simulink model "SHRKIM002_Dubins"  (R2026a)
settings: Solver=VariableStepAuto  StopTime=inf  MaxStep=0.04
InitFcn:
  | % Robot params
  | r_w = (67.60 / 2) / 1000; % wheel radius in m
  | d = (83 + 12.5 + 12.5) / 1000; % wheel centre-centre distance (width)
  | a = 33.275 / 1000; % IMU to wheel axle distance
  | 
  | % Motor params
  | k = 0.0192;
  | tau = 0.1718;
  | k_bodge = 3;
  | tau_bodge = 0.4;
  | 
  | noiseScalar = 1;
  | 
  | %control loop update rate
  | dt_loop = 0.02;
  | dt_sim = 0.005;
  | dt_plot = 0.1;
  | 
  | waypoint_matrix = centerlineTrack('SaoPaulo.csv');
model workspace (MAT data in the model file):
  d = Simulink.Parameter
  d.Value = 0.108
  d.Complexity = 'real'
  d.Dimensions = [1 1]
  d.DataType = 'auto'
  dphi_limit = Simulink.Parameter
  dphi_limit.Value = 9.72
  dphi_limit.Complexity = 'real'
  dphi_limit.Dimensions = [1 1]
  dphi_limit.DataType = 'double'
  dt_sim = Simulink.Parameter
  dt_sim.Value = 0.02
  dt_sim.Complexity = 'real'
  dt_sim.Dimensions = [1 1]
  dt_sim.DataType = 'auto'
  l_robot = Simulink.Parameter
  l_robot.Value = 0.103
  l_robot.Complexity = 'real'
  l_robot.Dimensions = [1 1]
  l_robot.DataType = 'auto'
  m_robot = Simulink.Parameter
  m_robot.Value = 0.5
  m_robot.Complexity = 'real'
  m_robot.Dimensions = [1 1]
  m_robot.DataType = 'auto'
  mpc_comp = mpc
  mpc_comp.Ts = 0.02
  mpc_comp.PredictionHorizon = 25
  mpc_comp.ControlHorizon = 2
  mpc_comp.Model.Plant = ss
  mpc_comp.Model.Plant.InputName_ = ["Robot Navigation & Control/Mux(1)"; "Robot Navigation & Control/Mux(2)"]
  mpc_comp.Model.Plant.InputGroup_.Manipulated = [1 2]
  mpc_comp.Model.Plant.OutputName_ = ["Plant Error Dynamics/1"; "Plant Error Dynamics/2"]
  mpc_comp.Model.Plant.OutputGroup_.Measured = [1 2]
  mpc_comp.Model.Plant.Name_ = 'Linearization at model initial condition'
  mpc_comp.Model.Plant.IOSize_ = [2 2]
  mpc_comp.Model.Plant.Data_ = ltipack.ssdata
  mpc_comp.Model.Plant.Data_.StateName = ["Integrator"; "Integrator1"]
  mpc_comp.Model.Plant.Data_.StatePath = ["SHRKIM002_FYP/Robot Navigation & Control/Plant Error Dynamics/Integrator"; "SHRKIM002_FYP/Robot Navigation & Control/Plant Error Dynamics/Integrator1"]
  mpc_comp.Model.Plant.Data_.a = [1  0; 0.004  1]
  mpc_comp.Model.Plant.Data_.c = [0  1; 1  0]
  mpc_comp.Model.Plant.Data_.dx0 = [0; 0]
  mpc_comp.Model.Plant.Data_.x0 = [0; 0]
  mpc_comp.Model.Plant.Data_.b = [-0.00625925925926  0.00625925925926; -1.25185185185e-05  1.25185185185e-05]
  mpc_comp.Model.Plant.Data_.d = [0  0; 0  0]
  mpc_comp.Model.Plant.Data_.u0 = [0; 0]
  mpc_comp.Model.Plant.Data_.y0 = [0; 0]
  mpc_comp.Model.Plant.Data_.Delay.Input = [0; 0]
  mpc_comp.Model.Plant.Data_.Delay.Output = [0; 0]
  mpc_comp.Model.Plant.Data_.Delay.Internal = []
  mpc_comp.Model.Plant.Data_.Ts = 0.02
  mpc_comp.Model.Disturbance = []
  mpc_comp.Model.Noise = []
  mpc_comp.Model.Nominal.X = [0; 0]
  mpc_comp.Model.Nominal.DX = [0; 0]
  mpc_comp.Model.Nominal.U = [0; 0]
  mpc_comp.Model.Nominal.Y = [0; 0]
  mpc_comp.ManipulatedVariables(1).Min = -9.72
  mpc_comp.ManipulatedVariables(1).Max = 9.72
  mpc_comp.ManipulatedVariables(1).MinECR = 0
  mpc_comp.ManipulatedVariables(1).MaxECR = 0
  mpc_comp.ManipulatedVariables(1).RateMin = -Inf
  mpc_comp.ManipulatedVariables(1).RateMax = Inf
  mpc_comp.ManipulatedVariables(1).RateMinECR = 0
  mpc_comp.ManipulatedVariables(1).RateMaxECR = 0
  mpc_comp.ManipulatedVariables(1).Target = 'nominal'
  mpc_comp.ManipulatedVariables(1).Name = 'Robot Navigation & Control/Mux(1)'
  mpc_comp.ManipulatedVariables(1).Units = ''
  mpc_comp.ManipulatedVariables(1).ScaleFactor = 1
  mpc_comp.ManipulatedVariables(1).Type = 'continuous'
  mpc_comp.ManipulatedVariables(2).Min = -9.72
  mpc_comp.ManipulatedVariables(2).Max = 9.72
  mpc_comp.ManipulatedVariables(2).MinECR = 0
  mpc_comp.ManipulatedVariables(2).MaxECR = 0
  mpc_comp.ManipulatedVariables(2).RateMin = -Inf
  mpc_comp.ManipulatedVariables(2).RateMax = Inf
  mpc_comp.ManipulatedVariables(2).RateMinECR = 0
  mpc_comp.ManipulatedVariables(2).RateMaxECR = 0
  mpc_comp.ManipulatedVariables(2).Target = 'nominal'
  mpc_comp.ManipulatedVariables(2).Name = 'Robot Navigation & Control/Mux(2)'
  mpc_comp.ManipulatedVariables(2).Units = ''
  mpc_comp.ManipulatedVariables(2).ScaleFactor = 1
  mpc_comp.ManipulatedVariables(2).Type = 'continuous'
  mpc_comp.OutputVariables(1).Min = -0.235
  mpc_comp.OutputVariables(1).Max = 0.235
  mpc_comp.OutputVariables(1).MinECR = 1
  mpc_comp.OutputVariables(1).MaxECR = 1
  mpc_comp.OutputVariables(1).Name = 'Plant Error Dynamics/1'
  mpc_comp.OutputVariables(1).Units = ''
  mpc_comp.OutputVariables(1).ScaleFactor = 1
  mpc_comp.OutputVariables(2).Min = -0.5236
  mpc_comp.OutputVariables(2).Max = 0.5236
  mpc_comp.OutputVariables(2).MinECR = 1
  mpc_comp.OutputVariables(2).MaxECR = 1
  mpc_comp.OutputVariables(2).Name = 'Plant Error Dynamics/2'
  mpc_comp.OutputVariables(2).Units = ''
  mpc_comp.OutputVariables(2).ScaleFactor = 1
  mpc_comp.Weights.ManipulatedVariables = [0.05 0.05]
  mpc_comp.Weights.ManipulatedVariablesRate = [0.1 0.1]
  mpc_comp.Weights.OutputVariables = [0.7 0.5]
  mpc_comp.Weights.ECR = 100000
  mpc_comp.Optimizer.OptimizationType = 'QP'
  mpc_comp.Optimizer.Solver = 'active-set'
  mpc_comp.Optimizer.SolverOptions = mpc.solver.options.qp.ActiveSet
  mpc_comp.Optimizer.SolverOptions.SolverName = 'ActiveSet'
  mpc_comp.Optimizer.MinOutputECR = 0
  mpc_comp.Optimizer.UseSuboptimalSolution = 0
  mpc_comp.Optimizer.CustomSolver = 0
  mpc_comp.Optimizer.CustomSolverCodeGen = 0
  mpc_comp.History = [2026 10 10 3 50 16.273]
  mpc_comp.MPCData = mpcdata
  mpc_comp.MPCData.IsDirty = 1
  mpc_comp.MPCData.Ts = 0.02
  mpc_comp.MPCData.p = 25
  mpc_comp.MPCData.m = 2
  mpc_comp.MPCData.UseActiveSetSolver = 1
  mpc_comp.MPCData.UseSuboptimalSolution = 0
  mpc_comp.MPCData.CustomSolver = 0
  mpc_comp.MPCData.CustomSolverCodeGen = 0
  mpc_comp.MPCData.IsCustomEstimation = 1
  mpc_comp.MPCData.Uscale = [1; 1]
  mpc_comp.MPCData.Yscale = [1; 1]
  mpc_comp.MPCData.mvindex = [1; 2]
  mpc_comp.MPCData.myindex = [1; 2]
  mpc_comp.MPCData.ASOptions.MaxIterations = 120
  mpc_comp.MPCData.ASOptions.ConstraintTolerance = 1e-06
  mpc_comp.MPCData.ASOptions.UseWarmStart = 1
  mpc_comp.MPCData.IPOptions.MaxIterations = 50
  mpc_comp.MPCData.IPOptions.ConstraintTolerance = 1e-06
  mpc_comp.MPCData.IPOptions.OptimalityTolerance = 1e-06
  mpc_comp.MPCData.IPOptions.ComplementarityTolerance = 1e-08
  mpc_comp.MPCData.IPOptions.StepTolerance = 1e-08
  mpc_comp.MPCData.ADOptions.AbsoluteTolerance = 0.001
  mpc_comp.MPCData.ADOptions.RelativeTolerance = 0.001
  mpc_comp.MPCData.ADOptions.MaxIterations = 1000
  mpc_comp.MPCData.ADOptions.RelaxationParameter = 1.6
  mpc_comp.MPCData.ADOptions.PenaltyParameter = 0.1
  mpc_comp.MPCData.ADOptions.StepSize = 1e-06
  mpc_comp.MPCData.ADOptions.PrimalInfeasibilityTolerance = 0.0001
  mpc_comp.MPCData.ADOptions.DualInfeasibilityTolerance = 0.0001
  mpc_comp.MPCData.ADOptions.EnablePolish = 0
  mpc_comp.MPCData.ADOptions.PolishRegularization = 1e-06
  mpc_comp.MPCData.ADOptions.PolishTolerance = 1e-08
  mpc_comp.MPCData.ADOptions.PolishMaxIterations = 3
  mpc_comp.MPCData.MIQPOptions.MaxIterations = 1000
  mpc_comp.MPCData.MIQPOptions.ConstraintTolerance = 1e-06
  mpc_comp.MPCData.MIQPOptions.UseWarmStart = 0
  mpc_comp.MPCData.MIQPOptions.DiscreteConstraintTolerance = 1e-06
  mpc_comp.MPCData.MIQPOptions.RoundingAtRootNode = 1
  mpc_comp.MPCData.MIQPOptions.MaxPendingNodes = 1000
  mpc_comp.IsEmpty = 0
  mpc_comp.OldOVIntegrator = {[]; []}
  mpc_comp.EstGain = 'custom'
  mpc_comp.OutDistModel = tf
  mpc_comp.OutDistModel.IOSize_ = [2 1]
  mpc_comp.OutDistModel.Data_ = ltipack.tfdata
  mpc_comp.OutDistModel.Data_.num = {0; 0}
  mpc_comp.OutDistModel.Data_.den = {1; 1}
  mpc_comp.OutDistModel.Data_.Delay.Input = 0
  mpc_comp.OutDistModel.Data_.Delay.Output = [0; 0]
  mpc_comp.OutDistModel.Data_.Delay.IO = [0; 0]
  mpc_comp.OutDistModel.Data_.Ts = 0
  mpc_comp.Version = '26.1'
  nlobj : nlmpc (value not decoded)
  no_points = Simulink.Parameter
  no_points.Value = 3000
  no_points.Complexity = 'real'
  no_points.Dimensions = [1 1]
  no_points.DataType = 'auto'
  r_w = Simulink.Parameter
  r_w.Value = 0.0338
  r_w.Complexity = 'real'
  r_w.Dimensions = [1 1]
  r_w.DataType = 'double'
  rho_min = Simulink.Parameter
  rho_min.Value = 0.2
  rho_min.Complexity = 'real'
  rho_min.Dimensions = [1 1]
  rho_min.DataType = 'auto'
  robot_half_w = Simulink.Parameter
  robot_half_w.Value = 0.065
  robot_half_w.Complexity = 'real'
  robot_half_w.Dimensions = [1 1]
  robot_half_w.DataType = 'auto'
  sample_f = Simulink.Parameter
  sample_f.Value = 50
  sample_f.Complexity = 'real'
  sample_f.Dimensions = [1 1]
  sample_f.DataType = 'auto'
  track_width = Simulink.Parameter
  track_width.Value = 0.6
  track_width.Complexity = 'real'
  track_width.Dimensions = [1 1]
  track_width.DataType = 'auto'
  waypoint_gain = Simulink.Parameter
  waypoint_gain.Value = 0.025
  waypoint_gain.Complexity = 'real'
  waypoint_gain.Dimensions = [1 1]
  waypoint_gain.DataType = 'auto'
values from neighbouring files (symbols this model uses):
  dphi_limit = 9.72    [controlNMPC.m]
undefined symbols (not defined in the file or in its folder): DiscIntNeverNeededParam
libraries: simulink x12, dspstat3 x6, slpidlib x2, mpclib x2, robotalgslib x1
(part 1 of 2)
settings Model: Creator=dylan  LastModifiedBy=Kim
settings SolverCC: DecoupledContinuousIntegration=on
settings SimscapeCC: SimscapeNominalValues="[{\"value\":\"1\",\"unit\":\"A\"},{\"value\":\"1\",\"unit\":\"bar\"},{\"value\":\"1\",\"unit\":\"cm^2\"},{\"value\":\"1\",\"unit\":\"cm^3/s\"},{\"value\":\"1\",\"unit\":\"kJ/kg\"},{\"value\":\"1\",\"unit\":\"kW\"},{\"value\":\"1\",\"unit\":\"l\"},{\"value\":\"1\",\"unit\":\"N\"},{\"value\":\"1\",\"unit\":\"N*m\"},{\"value\":\"1\",\"unit\":\"V\"}]"  SimscapeLogType=none  SimscapeLogDataHistory=5000.0

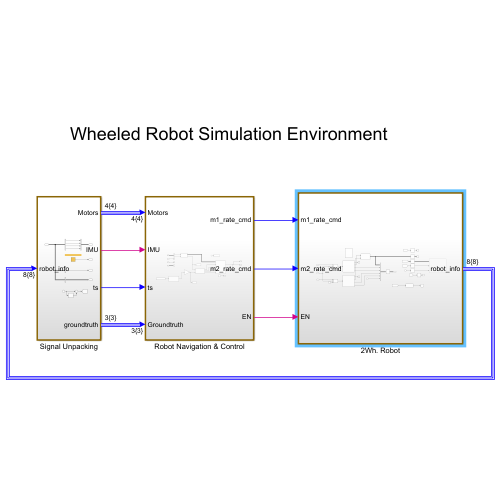
[thumbnail: Simulink's stored preview of the top-level diagram]
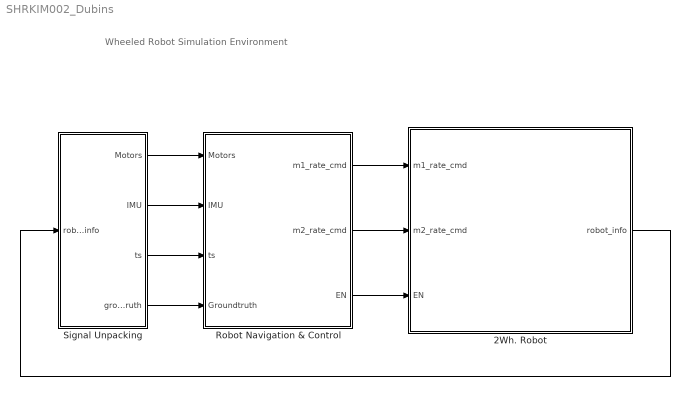
== system SHRKIM002_Dubins ==
  note: Wheeled Robot Simulation Environment
  2Wh. Robot : Subsystem
  Robot Navigation & Control : Subsystem
  Signal Unpacking : Subsystem
  wires:
  Robot Navigation & Control/1(m1_rate_cmd) -> 2Wh. Robot/1(m1_rate_cmd)
  Robot Navigation & Control/2(m2_rate_cmd) -> 2Wh. Robot/2(m2_rate_cmd)
  Robot Navigation & Control/3(EN) -> 2Wh. Robot/3(EN)
  Signal Unpacking/1(Motors) -> Robot Navigation & Control/1(Motors)
  Signal Unpacking/2(IMU) -> Robot Navigation & Control/2(IMU)
  Signal Unpacking/3(ts) -> Robot Navigation & Control/3(ts)
  Signal Unpacking/4(groundtruth) -> Robot Navigation & Control/4(Groundtruth)
  2Wh. Robot/1(robot_info) -> Signal Unpacking/1(robot_info)

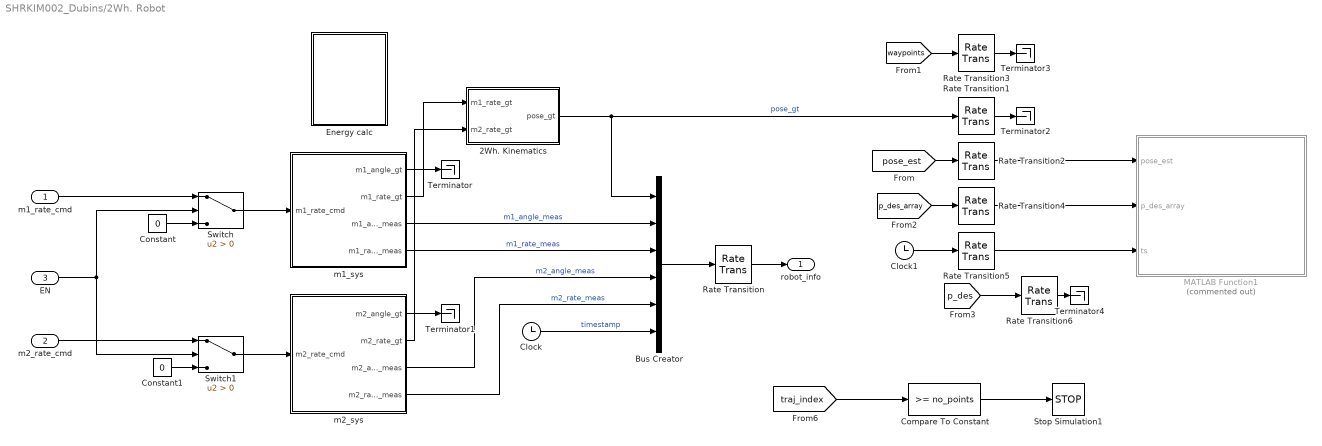
== system SHRKIM002_Dubins/2Wh. Robot ==
  m1_rate_cmd : Inport
  m2_rate_cmd : Inport  Port=2
  EN : Inport  Port=3
  2Wh. Kinematics : Subsystem
  Bus Creator : BusCreator  Inputs=6
  Clock : Clock
  Clock1 : Clock
  Compare To Constant : simulink/Logic and Bit Operations/Compare To Constant  relop=>=  const=no_points  OutDataTypeStr=boolean
  Constant : Constant  Value=0
  Constant1 : Constant  Value=0
  Energy calc : Subsystem
  MATLAB Function1 : MATLAB Function  Commented=on  TreatAsAtomicUnit=on
  Rate Transition : RateTransition  OutPortSampleTime=dt_loop
  Rate Transition1 : RateTransition  OutPortSampleTime=dt_plot
  Rate Transition2 : RateTransition  Deterministic=off  OutPortSampleTime=dt_plot
  Rate Transition3 : RateTransition  Deterministic=off  OutPortSampleTime=dt_plot
  Rate Transition4 : RateTransition  Deterministic=off  OutPortSampleTime=dt_plot
  Rate Transition5 : RateTransition  OutPortSampleTime=dt_plot
  Rate Transition6 : RateTransition  OutPortSampleTime=dt_plot
  Stop Simulation1 : Stop
  Switch : Switch  Criteria=u2 > Threshold  SaturateOnIntegerOverflow=off  InputSameDT=off
  Switch1 : Switch  Criteria=u2 > Threshold  SaturateOnIntegerOverflow=off  InputSameDT=off
  Terminator{,1..4} (5 alike) : Terminator
  m1_sys : Subsystem
  m2_sys : Subsystem
  robot_info : Outport
  wires:
  2Wh. Kinematics/1(pose_gt) -> Bus Creator/1, Rate Transition1/1  "pose_gt"
  m1_rate_cmd/1 -> Switch/1
  EN/1 -> Switch/2, Switch1/2
  m2_rate_cmd/1 -> Switch1/1
  Constant/1 -> Switch/3
  Constant1/1 -> Switch1/3
  Switch/1 -> m1_sys/1(m1_rate_cmd)
  m1_sys/1(m1_angle_gt) -> Terminator/1
  m1_sys/2(m1_rate_gt) -> 2Wh. Kinematics/1(m1_rate_gt)
  Switch1/1 -> m2_sys/1(m2_rate_cmd)
  m2_sys/1(m2_angle_gt) -> Terminator1/1
  m1_sys/3(m1_angle_meas) -> Bus Creator/2  "m1_angle_meas"
  m1_sys/4(m1_rate_meas) -> Bus Creator/3  "m1_rate_meas"
  m2_sys/3(m2_angle_meas) -> Bus Creator/4  "m2_angle_meas"
  m2_sys/4(m2_rate_meas) -> Bus Creator/5  "m2_rate_meas"
  Bus Creator/1 -> Rate Transition/1
  Rate Transition/1 -> robot_info/1
  Clock/1 -> Bus Creator/6  "timestamp"
  [pose_est] -> Rate Transition2/1
  Rate Transition2/1 -> MATLAB Function1/1(pose_est)
  m2_sys/2(m2_rate_gt) -> 2Wh. Kinematics/2(m2_rate_gt)
  [waypoints] -> Rate Transition3/1
  [p_des_array] -> Rate Transition4/1
  Rate Transition4/1 -> MATLAB Function1/2(p_des_array)
  Clock1/1 -> Rate Transition5/1
  Rate Transition5/1 -> MATLAB Function1/3(ts)
  [p_des] -> Rate Transition6/1
  Rate Transition6/1 -> Terminator4/1
  Rate Transition1/1 -> Terminator2/1
  Rate Transition3/1 -> Terminator3/1
  [traj_index] -> Compare To Constant/1
  Compare To Constant/1 -> Stop Simulation1/1

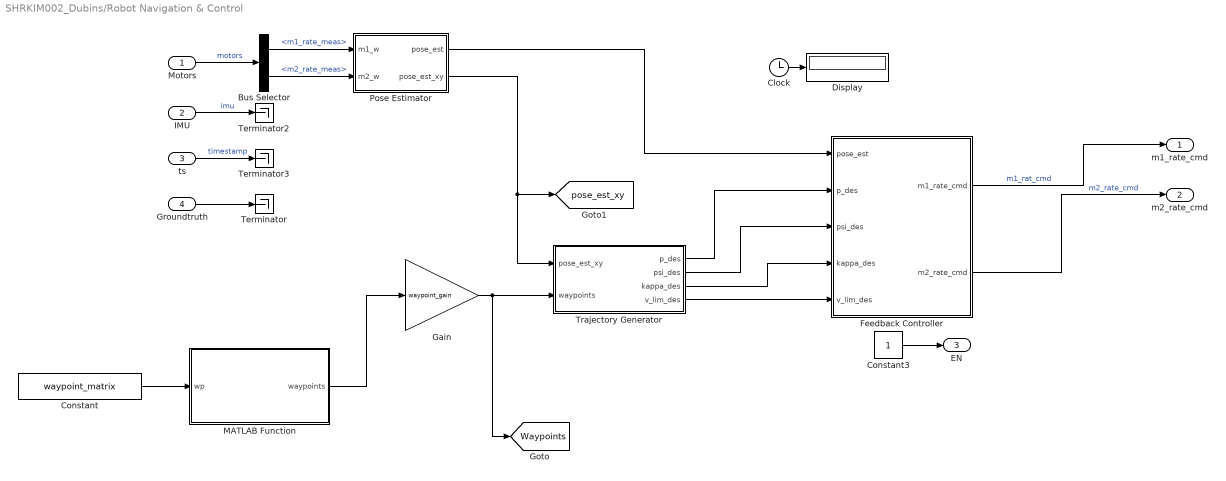
== system SHRKIM002_Dubins/Robot Navigation & Control ==
  Motors : Inport
  IMU : Inport  Port=2
  ts : Inport  Port=3
  Groundtruth : Inport  Port=4
  Bus Selector : BusSelector  OutputSignals=m1_rate_meas,m2_rate_meas
  Clock : Clock
  Constant : Constant  Value=waypoint_matrix
  Constant3 : Constant
  Display : Display
  Feedback Controller : Subsystem  Variant=on  VariantControlMode=label  LabelModeActiveChoice=LMPC
  Gain : Gain  Gain=waypoint_gain
  MATLAB Function : MATLAB Function  TreatAsAtomicUnit=on
  Pose Estimator : Subsystem
  Terminator : Terminator
  Terminator2 : Terminator
  Terminator3 : Terminator
  Trajectory Generator : Subsystem
  m1_rate_cmd : Outport
  m2_rate_cmd : Outport  Port=2
  EN : Outport  Port=3
  tag scope: Waypoints=global, pose_est_xy=global
  wires:
  IMU/1 -> Terminator2/1  "imu"
  Groundtruth/1 -> Terminator/1
  Constant3/1 -> EN/1
  Motors/1 -> Bus Selector/1  "motors"
  ts/1 -> Terminator3/1  "timestamp"
  Bus Selector/1 -> Pose Estimator/1(m1_w)  "<m1_rate_meas>"
  Bus Selector/2 -> Pose Estimator/2(m2_w)  "<m2_rate_meas>"
  Gain/1 -> [Waypoints], Trajectory Generator/2(waypoints)
  Trajectory Generator/1(p_des) -> Feedback Controller/2(p_des)
  Pose Estimator/2(pose_est_xy) -> Trajectory Generator/1(pose_est_xy), [pose_est_xy]
  Feedback Controller/2(m2_rate_cmd) -> m2_rate_cmd/1  "m2_rate_cmd"
  Feedback Controller/1(m1_rate_cmd) -> m1_rate_cmd/1  "m1_rat_cmd"
  Trajectory Generator/2(psi_des) -> Feedback Controller/3(psi_des)
  Trajectory Generator/3(kappa_des) -> Feedback Controller/4(kappa_des)
  Pose Estimator/1(pose_est) -> Feedback Controller/1(pose_est)
  MATLAB Function/1(waypoints) -> Gain/1
  Constant/1 -> MATLAB Function/1(wp)
  Clock/1 -> Display/1
  Trajectory Generator/4(v_lim_des) -> Feedback Controller/5(v_lim_des)

== system SHRKIM002_Dubins/Signal Unpacking ==
  note: Not yet implemented in sim
  robot_info : Inport
  Bus Creator : BusCreator  Inputs=4
  Bus Selector : BusSelector  OutputSignals=m1_angle_meas,m1_rate_meas,m2_angle_meas,m2_rate_meas
  Bus Selector1 : BusSelector  OutputSignals=timestamp
  Bus Selector2 : BusSelector  OutputSignals=pose_gt
  Clock : Clock
  Constant2 : Constant  Value=0
  Delay One Step : Delay  DelayLength=1
  Sum : Sum  Inputs=|+-
  Motors : Outport
  IMU : Outport  Port=2
  ts : Outport  Port=3
  groundtruth : Outport  Port=4
  tag scope: dT=global
  wires:
  Constant2/1 -> IMU/1
  Bus Selector/1 -> Bus Creator/1  "<m1_angle_meas>"
  Bus Selector/2 -> Bus Creator/2  "<m1_rate_meas>"
  Bus Selector/3 -> Bus Creator/3  "<m2_angle_meas>"
  Bus Selector/4 -> Bus Creator/4  "<m2_rate_meas>"
  Bus Creator/1 -> Motors/1
  Bus Selector1/1 -> ts/1  "<timestamp>"
  Bus Selector2/1 -> groundtruth/1  "<pose_gt>"
  robot_info/1 -> Bus Selector1/1, Bus Selector2/1, Bus Selector/1
  Clock/1 -> Delay One Step/1, Sum/1
  Sum/1 -> [dT]
  Delay One Step/1 -> Sum/2

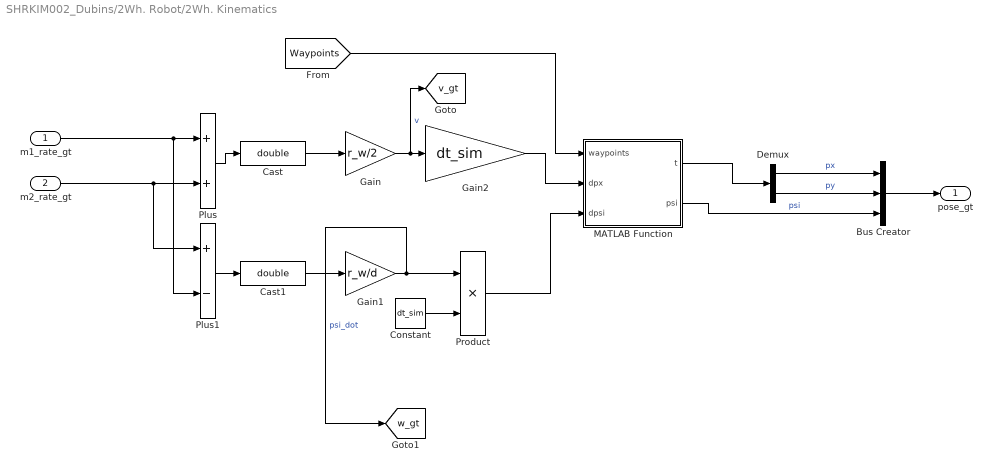
== system SHRKIM002_Dubins/2Wh. Robot/2Wh. Kinematics ==
  m1_rate_gt : Inport
  m2_rate_gt : Inport  Port=2
  Bus Creator : BusCreator  Inputs=3
  Cast : DataTypeConversion  OutDataTypeStr=double  SaturateOnIntegerOverflow=off  RndMeth=Floor
  Cast1 : DataTypeConversion  OutDataTypeStr=double  SaturateOnIntegerOverflow=off  RndMeth=Floor
  Constant : Constant  Value=dt_sim
  Demux : Demux  Outputs=2
  Gain : Gain  Gain=r_w/2
  Gain1 : Gain  Gain=r_w/d
  Gain2 : Gain  Gain=dt_sim
  MATLAB Function : MATLAB Function  TreatAsAtomicUnit=on
  Plus : Sum
  Plus1 : Sum  Inputs=+-
  Product : Product
  pose_gt : Outport
  tag scope: v_gt=global, w_gt=global
  wires:
  Plus/1 -> Cast/1
  Plus1/1 -> Cast1/1
  Cast1/1 -> Gain1/1
  Cast/1 -> Gain/1
  Bus Creator/1 -> pose_gt/1
  Gain1/1 -> [w_gt], Product/1  "psi_dot"
  Gain/1 -> [v_gt], Gain2/1  "v"
  Demux/1 -> Bus Creator/1  "px"
  Demux/2 -> Bus Creator/2  "py"
  MATLAB Function/1(t) -> Demux/1
  MATLAB Function/2(psi) -> Bus Creator/3  "psi"
  Product/1 -> MATLAB Function/3(dpsi)
  m1_rate_gt/1 -> Plus1/2, Plus/1
  m2_rate_gt/1 -> Plus1/1, Plus/2
  Gain2/1 -> MATLAB Function/2(dpx)
  Constant/1 -> Product/2
  [Waypoints] -> MATLAB Function/1(waypoints)

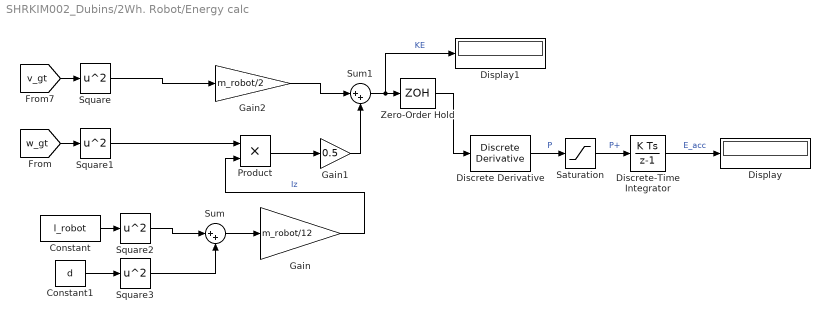
== system SHRKIM002_Dubins/2Wh. Robot/Energy calc ==
  Constant : Constant  Value=l_robot
  Constant1 : Constant  Value=d
  Discrete Derivative : simulink/Discrete/Discrete Derivative  gainval=1.0  ICPrevScaledInput=0.0  OutMin=[]  OutMax=[]  OutDataType=fixdt(1, 16)  OutScaling=2^-10  DoSatur=off
  Discrete-Time Integrator : DiscreteIntegrator  SampleTime=dt_sim  ICPrevOutput=DiscIntNeverNeededParam  ICPrevScaledInput=DiscIntNeverNeededParam
  Display : Display
  Display1 : Display
  Gain : Gain  Gain=m_robot/12
  Gain1 : Gain  Gain=0.5
  Gain2 : Gain  Gain=m_robot/2
  Product : Product
  Saturation : Saturate  UpperLimit=inf  LowerLimit=0
  Square{,1..3} (4 alike) : Math  Operator=square
  Sum : Sum  Inputs=|++
  Sum1 : Sum  Inputs=|++
  Zero-Order Hold : ZeroOrderHold  SampleTime=dt_sim
  wires:
  [v_gt] -> Square/1
  [w_gt] -> Square1/1
  Constant/1 -> Square2/1
  Constant1/1 -> Square3/1
  Square2/1 -> Sum/1
  Square3/1 -> Sum/2
  Sum/1 -> Gain/1
  Gain/1 -> Product/2  "Iz"
  Square1/1 -> Product/1
  Product/1 -> Gain1/1
  Square/1 -> Gain2/1
  Gain1/1 -> Sum1/2
  Gain2/1 -> Sum1/1
  Sum1/1 -> Display1/1, Zero-Order Hold/1  "KE"
  Zero-Order Hold/1 -> Discrete Derivative/1
  Discrete Derivative/1 -> Saturation/1  "P"
  Saturation/1 -> Discrete-Time Integrator/1  "P+"
  Discrete-Time Integrator/1 -> Display/1  "E_acc"

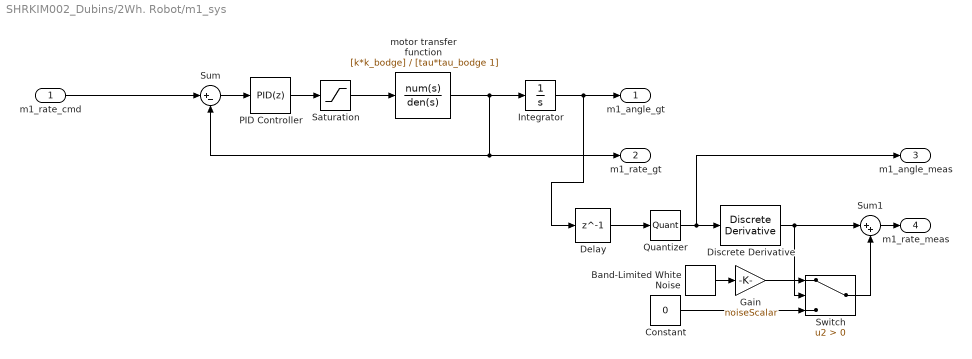
== system SHRKIM002_Dubins/2Wh. Robot/m1_sys ==
  m1_rate_cmd : Inport
  Band-Limited White Noise : simulink/Sources/Band-Limited White Noise  Cov=[0.001]  Ts=0.005  seed=[23341]
  Constant : Constant  Value=0
  Delay : Delay  DelayLength=1  SampleTime=0.01
  Discrete Derivative : simulink/Discrete/Discrete Derivative  gainval=1.0  ICPrevScaledInput=0.0  OutMin=[]  OutMax=[]  OutDataType=fixdt(1, 16)  OutScaling=2^-10  DoSatur=off
  Gain : Gain  Gain=noiseScalar
  Integrator : Integrator
  PID Controller : slpidlib/PID Controller  Controller=PID  Form=Parallel  TimeDomain=Discrete-time  UseExternalTs=off  SampleTime=0.01  IntegratorMethod=Forward Euler  FilterMethod=Forward Euler  ControllerParametersSource=internal  P=80  I=90  UseKiTs=off  D=0  UseExternalDerivativeSource=off  N=100  UseFilter=on  TunerSelectOption=Transfer Function Based (PID Tuner App)  InitialConditionSource=internal  InitialConditionForIntegrator=0  InitialConditionForFilter=0  DifferentiatorICPrevScaledInput=0  ExternalReset=none  TrackingMode=off  Kt=1  LimitOutput=off  SatLimitsSource=internal  UpperSaturationLimit=inf  LowerSaturationLimit=-inf  LinearizeAsGain=on  AntiWindupMode=none  Kb=1  LimitIntegrator=off  UpperIntegratorSaturationLimit=inf  LowerIntegratorSaturationLimit=-inf  POutMin=[]  POutMax=[]  IOutMin=[]  IOutMax=[]  DOutMin=[]  DOutMax=[]  NOutMin=[]  NOutMax=[]  SumOutMin=[]  SumOutMax=[]  SaturationOutMin=[]  SaturationOutMax=[]  PParamMin=[]  PParamMax=[]  IParamMin=[]  IParamMax=[]  DParamMin=[]  DParamMax=[]  NParamMin=[]  NParamMax=[]  KbParamMin=[]  KbParamMax=[]  KtParamMin=[]  KtParamMax=[]  KbOutMin=[]  KbOutMax=[]  KtOutMin=[]  KtOutMax=[]  IntegratorOutMin=[]  IntegratorOutMax=[]  FilterOutMin=[]  FilterOutMax=[]  SumI1OutMin=[]  SumI1OutMax=[]  SumI2OutMin=[]  SumI2OutMax=[]  SumI3OutMin=[]  SumI3OutMax=[]  SumI4OutMin=[]  SumI4OutMax=[]  SumDOutMin=[]  SumDOutMax=[]  DifferentiatorOutMin=[]  DifferentiatorOutMax=[]  FilterDiffOutCoefMin=[]  FilterDiffOutCoefMax=[]  ReciprocalOutMin=[]  ReciprocalOutMax=[]  SumDenOutMin=[]  SumDenOutMax=[]  SumNumOutMin=[]  SumNumOutMax=[]  DivideOutMin=[]  DivideOutMax=[]  UdiffTsProdOutMin=[]  UdiffTsProdOutMax=[]  NTsProdOutMin=[]  NTsProdOutMax=[]  UintegralTsProdOutMin=[]  UintegralTsProdOutMax=[]  UngainTsProdOutMin=[]  UngainTsProdOutMax=[]  ClampingZeroOutDataTypeStr=Inherit: Inherit via back propagation  ClampingZeroOutMin=[]  ClampingZeroOutMax=[]  FilterDenConstantOutDataTypeStr=Inherit: Inherit via back propagation  FilterDenConstantOutMin=[]  FilterDenConstantOutMax=[]  PCopyOutDataTypeStr=Inherit: Inherit via back propagation  PCopyOutMin=[]  PCopyOutMax=[]  NCopyOutDataTypeStr=Inherit: Inherit via back propagation  NCopyOutMin=[]  NCopyOutMax=[]  IntegratorContinuousStateAttributes=''  IntegratorStateMustResolveToSignalObject=off  IntegratorRTWStateStorageClass=Auto  FilterContinuousStateAttributes=''  FilterStateMustResolveToSignalObject=off  FilterRTWStateStorageClass=Auto  ParallelPVariant=InternalParameters  IdealPVariant=Disabled  IVariant=InternalParameters  DVariant=InternalParameters  IntegratorVariant=Discrete  SatVariant=Disabled  AWVariant=Passthrough  PCopyVariant=Disabled  TRVariant=Disabled  FdbkBlocksVariant=Forward  IdealPFdbkVariant=Disabled  SatFdbkVariant=Disabled  DerivativeFilterVariant=ForwardEulerFilter  NVariant=InternalParameters  NCopyVariant=Disabled  FilterICVariant=InternalICsFilter  IntegratorICVariant=InternalICs  ExternalResetVariant=Disabled  TRSumVariant=Passthrough  SumFdbkVariant=Disabled  SumVariant=Sum_PID  TsampFilterVariant=InternalTs  TsampNgainVariant=Passthrough  TsampIntegralVariant=Disabled_SignalSpec  ExternalSaturationOutDataTypeStr=Inherit: Same as second input  DerivativeSourceVariant=ErrorSignal  PreIntVariant=InternalPreInt
  Quantizer : Quantizer  QuantizationInterval=2*pi/(540*8)  LinearizeAsGain=off
  Saturation : Saturate  UpperLimit=255  LowerLimit=-255
  Sum : Sum  Inputs=|+-
  Sum1 : Sum  Inputs=|++
  Switch : Switch  Criteria=u2 > Threshold  SaturateOnIntegerOverflow=off  InputSameDT=off
  motor transfer function : TransferFcn  Numerator=[k*k_bodge]  Denominator=[tau*tau_bodge 1]
  m1_angle_gt : Outport
  m1_rate_gt : Outport  Port=2
  m1_angle_meas : Outport  Port=3
  m1_rate_meas : Outport  Port=4
  wires:
  Band-Limited White Noise/1 -> Gain/1
  motor transfer function/1 -> Integrator/1, m1_rate_gt/1, Sum/2
  Sum/1 -> PID Controller/1
  Discrete Derivative/1 -> Switch/2, Sum1/1
  Integrator/1 -> m1_angle_gt/1, Delay/1
  Delay/1 -> Quantizer/1
  PID Controller/1 -> Saturation/1
  Quantizer/1 -> m1_angle_meas/1, Discrete Derivative/1
  Sum1/1 -> m1_rate_meas/1
  Saturation/1 -> motor transfer function/1
  Gain/1 -> Switch/1
  Switch/1 -> Sum1/2
  Constant/1 -> Switch/3
  m1_rate_cmd/1 -> Sum/1

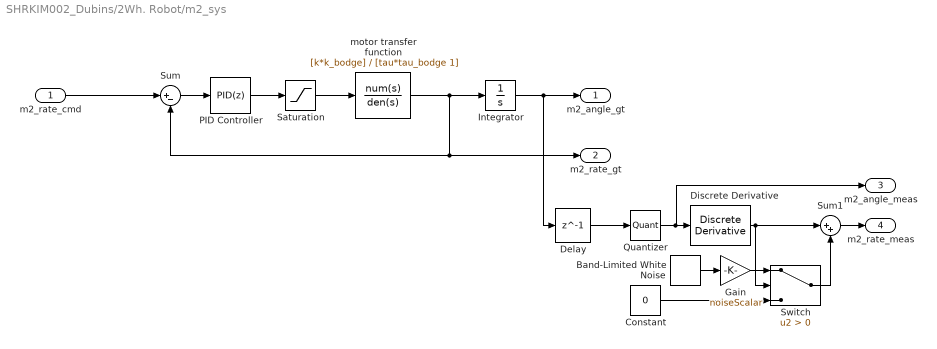
== system SHRKIM002_Dubins/2Wh. Robot/m2_sys ==
  m2_rate_cmd : Inport
  Band-Limited White Noise : simulink/Sources/Band-Limited White Noise  Cov=[0.001]  Ts=0.005  seed=[23341]
  Constant : Constant  Value=0
  Delay : Delay  DelayLength=1  SampleTime=0.01
  Discrete Derivative : simulink/Discrete/Discrete Derivative  gainval=1.0  ICPrevScaledInput=0.0  OutMin=[]  OutMax=[]  OutDataType=fixdt(1, 16)  OutScaling=2^-10  DoSatur=off
  Gain : Gain  Gain=noiseScalar
  Integrator : Integrator
  PID Controller : slpidlib/PID Controller  Controller=PID  Form=Parallel  TimeDomain=Discrete-time  UseExternalTs=off  SampleTime=0.01  IntegratorMethod=Forward Euler  FilterMethod=Forward Euler  ControllerParametersSource=internal  P=80  I=90  UseKiTs=off  D=0  UseExternalDerivativeSource=off  N=100  UseFilter=on  TunerSelectOption=Transfer Function Based (PID Tuner App)  InitialConditionSource=internal  InitialConditionForIntegrator=0  InitialConditionForFilter=0  DifferentiatorICPrevScaledInput=0  ExternalReset=none  TrackingMode=off  Kt=1  LimitOutput=off  SatLimitsSource=internal  UpperSaturationLimit=inf  LowerSaturationLimit=-inf  LinearizeAsGain=on  AntiWindupMode=none  Kb=1  LimitIntegrator=off  UpperIntegratorSaturationLimit=inf  LowerIntegratorSaturationLimit=-inf  POutMin=[]  POutMax=[]  IOutMin=[]  IOutMax=[]  DOutMin=[]  DOutMax=[]  NOutMin=[]  NOutMax=[]  SumOutMin=[]  SumOutMax=[]  SaturationOutMin=[]  SaturationOutMax=[]  PParamMin=[]  PParamMax=[]  IParamMin=[]  IParamMax=[]  DParamMin=[]  DParamMax=[]  NParamMin=[]  NParamMax=[]  KbParamMin=[]  KbParamMax=[]  KtParamMin=[]  KtParamMax=[]  KbOutMin=[]  KbOutMax=[]  KtOutMin=[]  KtOutMax=[]  IntegratorOutMin=[]  IntegratorOutMax=[]  FilterOutMin=[]  FilterOutMax=[]  SumI1OutMin=[]  SumI1OutMax=[]  SumI2OutMin=[]  SumI2OutMax=[]  SumI3OutMin=[]  SumI3OutMax=[]  SumI4OutMin=[]  SumI4OutMax=[]  SumDOutMin=[]  SumDOutMax=[]  DifferentiatorOutMin=[]  DifferentiatorOutMax=[]  FilterDiffOutCoefMin=[]  FilterDiffOutCoefMax=[]  ReciprocalOutMin=[]  ReciprocalOutMax=[]  SumDenOutMin=[]  SumDenOutMax=[]  SumNumOutMin=[]  SumNumOutMax=[]  DivideOutMin=[]  DivideOutMax=[]  UdiffTsProdOutMin=[]  UdiffTsProdOutMax=[]  NTsProdOutMin=[]  NTsProdOutMax=[]  UintegralTsProdOutMin=[]  UintegralTsProdOutMax=[]  UngainTsProdOutMin=[]  UngainTsProdOutMax=[]  ClampingZeroOutDataTypeStr=Inherit: Inherit via back propagation  ClampingZeroOutMin=[]  ClampingZeroOutMax=[]  FilterDenConstantOutDataTypeStr=Inherit: Inherit via back propagation  FilterDenConstantOutMin=[]  FilterDenConstantOutMax=[]  PCopyOutDataTypeStr=Inherit: Inherit via back propagation  PCopyOutMin=[]  PCopyOutMax=[]  NCopyOutDataTypeStr=Inherit: Inherit via back propagation  NCopyOutMin=[]  NCopyOutMax=[]  IntegratorContinuousStateAttributes=''  IntegratorStateMustResolveToSignalObject=off  IntegratorRTWStateStorageClass=Auto  FilterContinuousStateAttributes=''  FilterStateMustResolveToSignalObject=off  FilterRTWStateStorageClass=Auto  ParallelPVariant=InternalParameters  IdealPVariant=Disabled  IVariant=InternalParameters  DVariant=InternalParameters  IntegratorVariant=Discrete  SatVariant=Disabled  AWVariant=Passthrough  PCopyVariant=Disabled  TRVariant=Disabled  FdbkBlocksVariant=Forward  IdealPFdbkVariant=Disabled  SatFdbkVariant=Disabled  DerivativeFilterVariant=ForwardEulerFilter  NVariant=InternalParameters  NCopyVariant=Disabled  FilterICVariant=InternalICsFilter  IntegratorICVariant=InternalICs  ExternalResetVariant=Disabled  TRSumVariant=Passthrough  SumFdbkVariant=Disabled  SumVariant=Sum_PID  TsampFilterVariant=InternalTs  TsampNgainVariant=Passthrough  TsampIntegralVariant=Disabled_SignalSpec  ExternalSaturationOutDataTypeStr=Inherit: Same as second input  DerivativeSourceVariant=ErrorSignal  PreIntVariant=InternalPreInt
  Quantizer : Quantizer  QuantizationInterval=2*pi/(540*8)  LinearizeAsGain=off
  Saturation : Saturate  UpperLimit=255  LowerLimit=-255
  Sum : Sum  Inputs=|+-
  Sum1 : Sum  Inputs=|++
  Switch : Switch  Criteria=u2 > Threshold  SaturateOnIntegerOverflow=off  InputSameDT=off
  motor transfer function : TransferFcn  Numerator=[k*k_bodge]  Denominator=[tau*tau_bodge 1]
  m2_angle_gt : Outport
  m2_rate_gt : Outport  Port=2
  m2_angle_meas : Outport  Port=3
  m2_rate_meas : Outport  Port=4
  wires:
  Band-Limited White Noise/1 -> Gain/1
  motor transfer function/1 -> Integrator/1, m2_rate_gt/1, Sum/2
  Sum/1 -> PID Controller/1
  PID Controller/1 -> Saturation/1
  Discrete Derivative/1 -> Sum1/1, Switch/2
  Integrator/1 -> m2_angle_gt/1, Delay/1
  Delay/1 -> Quantizer/1
  Saturation/1 -> motor transfer function/1
  Quantizer/1 -> m2_angle_meas/1, Discrete Derivative/1
  Sum1/1 -> m2_rate_meas/1
  Gain/1 -> Switch/1
  Switch/1 -> Sum1/2
  Constant/1 -> Switch/3
  m2_rate_cmd/1 -> Sum/1

== system SHRKIM002_Dubins/Robot Navigation & Control/Feedback Controller ==
  pose_est : Inport
  p_des : Inport  Port=2
  psi_des : Inport  Port=3
  kappa_des : Inport  Port=4
  v_lim_des : Inport  Port=5
  LMPC : Subsystem  VariantControl=LMPC
  NMPC : Subsystem  VariantControl=NMPC
  Pure Pursuit : Subsystem  VariantControl=Pure Pursuit
  m1_rate_cmd : Outport
  m2_rate_cmd : Outport  Port=2

== system SHRKIM002_Dubins/Robot Navigation & Control/Pose Estimator ==
  m1_w : Inport
  m2_w : Inport  Port=2
  Add : Sum
  Bus Creator : BusCreator  Inputs=3
  Gain : Gain  Gain=0.5
  Gain1 : Gain  Gain=r_w
  Gain2 : Gain  Gain=r_w
  Gain3 : Gain  Gain=1/d
  MATLAB Function : MATLAB Function  TreatAsAtomicUnit=on
  Subtract : Sum  Inputs=+-
  dT : Constant  Value=1/sample_f
  pose_est : Outport
  pose_est_xy : Outport  Port=2
  tag scope: pose_est=global
  wires:
  Bus Creator/1 -> pose_est/1, [pose_est]
  MATLAB Function/1(px_est) -> Bus Creator/1  "px_est"
  MATLAB Function/2(py_est) -> Bus Creator/2  "py_est"
  MATLAB Function/3(psi_est) -> Bus Creator/3  "psi_est"
  m1_w/1 -> Subtract/2, Add/1
  m2_w/1 -> Subtract/1, Add/2
  Add/1 -> Gain1/1
  Gain1/1 -> Gain/1
  Subtract/1 -> Gain2/1
  Gain2/1 -> Gain3/1
  Gain/1 -> MATLAB Function/1(v)  "v"
  Gain3/1 -> MATLAB Function/2(psi_dot)  "psi_dot"
  dT/1 -> MATLAB Function/3(dT)
  MATLAB Function/4(pose_est_xy) -> pose_est_xy/1
  [Waypoints] -> MATLAB Function/4(waypoints)

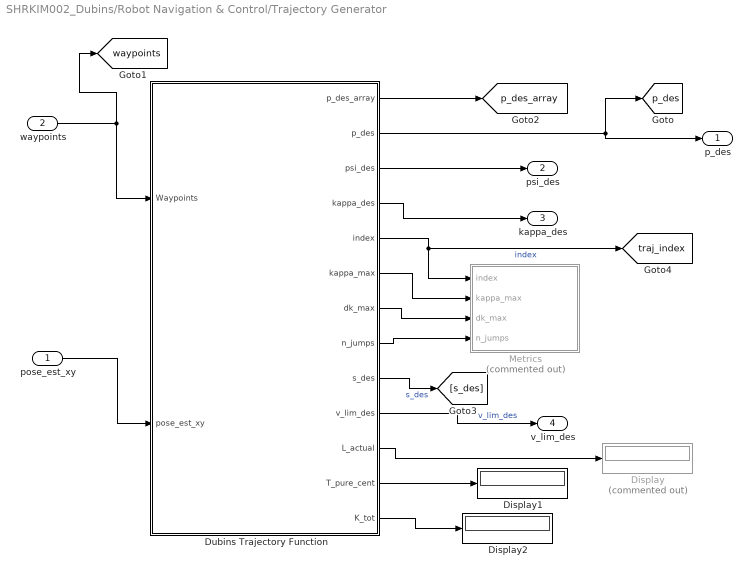
== system SHRKIM002_Dubins/Robot Navigation & Control/Trajectory Generator ==
  pose_est_xy : Inport
  waypoints : Inport  Port=2
  Display : Display  Commented=on
      settings: Decimation=3
  Display1 : Display
  Display2 : Display
  Dubins Trajectory Function : MATLAB Function  TreatAsAtomicUnit=on  SystemSampleTime=0.02
  Metrics : Subsystem  Commented=on
  p_des : Outport
  psi_des : Outport  Port=2
  kappa_des : Outport  Port=3
  v_lim_des : Outport  Port=4
  tag scope: p_des=global, p_des_array=global, traj_index=global, waypoints=global
  wires:
  waypoints/1 -> Dubins Trajectory Function/1(Waypoints), [waypoints]
  pose_est_xy/1 -> Dubins Trajectory Function/2(pose_est_xy)
  Dubins Trajectory Function/2(p_des) -> [p_des], p_des/1
  Dubins Trajectory Function/1(p_des_array) -> [p_des_array]
  Dubins Trajectory Function/3(psi_des) -> psi_des/1
  Dubins Trajectory Function/4(kappa_des) -> kappa_des/1
  Dubins Trajectory Function/5(index) -> [traj_index], Metrics/1(index)  "index"
  Dubins Trajectory Function/6(kappa_max) -> Metrics/2(kappa_max)
  Dubins Trajectory Function/7(dk_max) -> Metrics/3(dk_max)
  Dubins Trajectory Function/8(n_jumps) -> Metrics/4(n_jumps)
  Dubins Trajectory Function/10(v_lim_des) -> v_lim_des/1  "v_lim_des"
  Dubins Trajectory Function/9(s_des) -> [s_des]  "s_des"
  Dubins Trajectory Function/11(L_actual) -> Display/1
  Dubins Trajectory Function/13(K_tot) -> Display2/1
  Dubins Trajectory Function/12(T_pure_cent) -> Display1/1

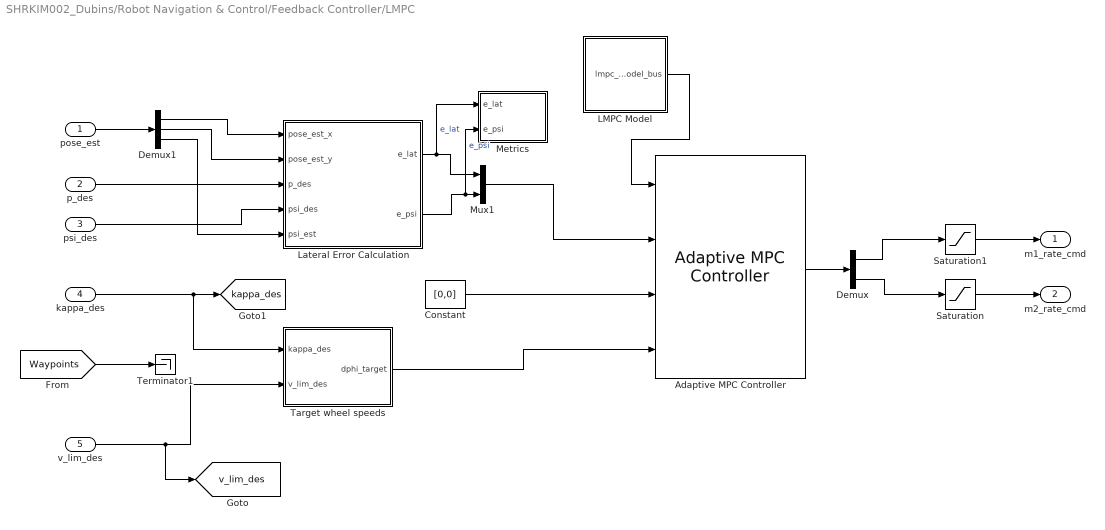
== system SHRKIM002_Dubins/Robot Navigation & Control/Feedback Controller/LMPC ==
  pose_est : Inport
  p_des : Inport  Port=2
  psi_des : Inport  Port=3
  kappa_des : Inport  Port=4
  v_lim_des : Inport  Port=5
  Adaptive MPC Controller : mpclib/Adaptive MPC Controller  SCDEnableBlockLinearizationSpecification=on  mpcobj=mpc_comp  enable_value=0  updateMPCinCallerWorkspace=on  md_inport=off  mv_inport=off  uref_inport=on  return_cost=off  return_mvseq=off  return_qpstatus=off  return_xseq=off  return_state=off  return_ovseq=off  state_inport=on  isltv_plant=off  umin_inport=off  umax_inport=off  ymin_inport=off  ymax_inport=off  cc_inport=off  ywt_inport=off  uwt_inport=off  duwt_inport=off  rhoeps_inport=off  pm_inport=off  MaximumP=10  HorizonChoice=FixedHorizon  BlockDataType=double  SampleTimeInherited=off  switch_inport=off
  Constant : Constant  Value=[0,0]  VectorParams1D=off
  Demux : Demux  Outputs=2
  Demux1 : Demux  Outputs=3
  LMPC Model : Subsystem
  Lateral Error Calculation : MATLAB Function  TreatAsAtomicUnit=on
  Metrics : Subsystem
  Mux1 : Mux  Inputs=2
  Saturation : Saturate  UpperLimit=dphi_limit  LowerLimit=-dphi_limit
  Saturation1 : Saturate  UpperLimit=dphi_limit  LowerLimit=-dphi_limit
  Target wheel speeds : Subsystem
  Terminator1 : Terminator
  m1_rate_cmd : Outport
  m2_rate_cmd : Outport  Port=2
  tag scope: kappa_des=global, v_lim_des=global
  wires:
  p_des/1 -> Lateral Error Calculation/3(p_des)
  psi_des/1 -> Lateral Error Calculation/4(psi_des)
  pose_est/1 -> Demux1/1
  Demux1/1 -> Lateral Error Calculation/1(pose_est_x)
  Demux1/2 -> Lateral Error Calculation/2(pose_est_y)
  Demux1/3 -> Lateral Error Calculation/5(psi_est)
  Lateral Error Calculation/1(e_lat) -> Metrics/1(e_lat), Mux1/1  "e_lat"
  Lateral Error Calculation/2(e_psi) -> Metrics/2(e_psi), Mux1/2  "e_psi"
  Mux1/1 -> Adaptive MPC Controller/2
  Constant/1 -> Adaptive MPC Controller/3
  [Waypoints] -> Terminator1/1
  Saturation/1 -> m2_rate_cmd/1
  Saturation1/1 -> m1_rate_cmd/1
  kappa_des/1 -> Target wheel speeds/1(kappa_des), [kappa_des]
  Target wheel speeds/1(dphi_target) -> Adaptive MPC Controller/4
  Adaptive MPC Controller/1 -> Demux/1
  Demux/1 -> Saturation1/1
  Demux/2 -> Saturation/1
  v_lim_des/1 -> [v_lim_des], Target wheel speeds/2(v_lim_des)
  LMPC Model/1(lmpc_model_bus) -> Adaptive MPC Controller/1

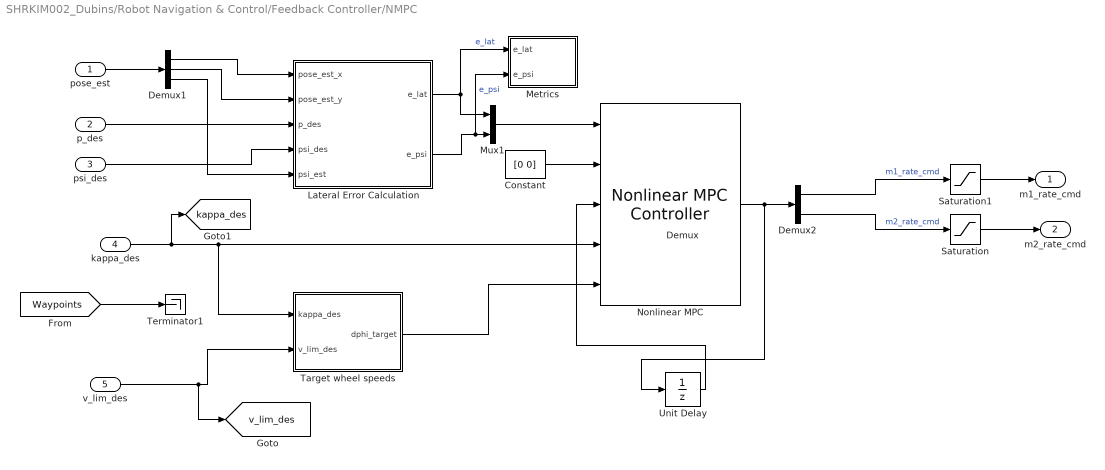
== system SHRKIM002_Dubins/Robot Navigation & Control/Feedback Controller/NMPC ==
  pose_est : Inport
  p_des : Inport  Port=2
  psi_des : Inport  Port=3
  kappa_des : Inport  Port=4
  v_lim_des : Inport  Port=5
  Constant : Constant  Value=[0 0]  VectorParams1D=off
  Demux : Demux  Outputs=2
  Demux1 : Demux  Outputs=3
  Demux2 : Demux  Outputs=2
  Lateral Error Calculation : MATLAB Function  TreatAsAtomicUnit=on
  Metrics : Subsystem
  Mux1 : Mux  Inputs=2
  Nonlinear MPC : mpclib/Nonlinear MPC Controller  nlmpcobj=nlobj  md_enabled=on  mvtarget_enabled=on  param_enabled=off  cost_enabled=off  mvseq_enabled=off  stateseq_enabled=off  ovseq_enabled=off  slack_enabled=off  status_enabled=off  ov_min=off  ov_max=off  mv_min=off  mv_max=off  mvrate_min=off  mvrate_max=off  state_min=off  state_max=off  ov_weight=off  mv_weight=off  mvrate_weight=off  ecr_weight=off  nlp_initialize=off  BlockDataType=double  UseObjectTs=on  UseMEX=off
  Saturation : Saturate  UpperLimit=dphi_limit  LowerLimit=-dphi_limit
  Saturation1 : Saturate  UpperLimit=dphi_limit  LowerLimit=-dphi_limit
  Target wheel speeds : Subsystem
  Terminator1 : Terminator
  Unit Delay : UnitDelay  InitialCondition=[0; 0]  SampleTime=-1
  m1_rate_cmd : Outport
  m2_rate_cmd : Outport  Port=2
  tag scope: kappa_des=global, v_lim_des=global
  wires:
  Demux1/1 -> Lateral Error Calculation/1(pose_est_x)
  psi_des/1 -> Lateral Error Calculation/4(psi_des)
  [Waypoints] -> Terminator1/1
  Demux1/3 -> Lateral Error Calculation/5(psi_est)
  Lateral Error Calculation/2(e_psi) -> Metrics/2(e_psi), Mux1/2  "e_psi"
  Demux2/1 -> Saturation1/1  "m1_rate_cmd"
  p_des/1 -> Lateral Error Calculation/3(p_des)
  Demux2/2 -> Saturation/1  "m2_rate_cmd"
  Lateral Error Calculation/1(e_lat) -> Metrics/1(e_lat), Mux1/1  "e_lat"
  pose_est/1 -> Demux1/1
  Demux1/2 -> Lateral Error Calculation/2(pose_est_y)
  Nonlinear MPC/1 -> Demux2/1, Unit Delay/1
  Mux1/1 -> Nonlinear MPC/1
  Constant/1 -> Nonlinear MPC/2
  Unit Delay/1 -> Nonlinear MPC/3
  Saturation/1 -> m2_rate_cmd/1
  Saturation1/1 -> m1_rate_cmd/1
  kappa_des/1 -> [kappa_des], Target wheel speeds/1(kappa_des), Nonlinear MPC/4
  Target wheel speeds/1(dphi_target) -> Nonlinear MPC/5
  v_lim_des/1 -> [v_lim_des], Target wheel speeds/2(v_lim_des)

== system SHRKIM002_Dubins/Robot Navigation & Control/Feedback Controller/Pure Pursuit ==
  pose_est : Inport
  p_des : Inport  Port=2
  psi_des : Inport  Port=3
  kappa_des : Inport  Port=4
  v_lim_des : Inport  Port=5
  Bus Selector : BusSelector  OutputSignals=px_est,py_est,psi_est
  Mux : Mux  Inputs=3
  Outer Wheel Limiter : Subsystem
  Pure Pursuit : robotalgslib/Pure Pursuit  DesiredLinearVelocityPort=on  DesiredLinearVelocity=0.2  MaxCurvature=6  LookaheadDistancePort=off  LookaheadDistance=0.2  TargetDirPort=off  SimulateUsing=Code generation
      settings: LibrarySourceBlock=robotmobilelib/Pure Pursuit
  Switches : Subsystem
  Terminator2 : Terminator
  Transpose : Math  Operator=transpose
  m1_rate_cmd : Outport
  m2_rate_cmd : Outport  Port=2
  wires:
  [p_des_array] -> Transpose/1
  Transpose/1 -> Pure Pursuit/2
  pose_est/1 -> Bus Selector/1
  Bus Selector/3 -> Switches/5(<psi_est>), Mux/3  "<psi_est>"
  Bus Selector/2 -> Switches/4(<py_est>), Mux/2  "<py_est>"
  Bus Selector/1 -> Switches/3(<px_est>), Mux/1  "<px_est>"
  Mux/1 -> Pure Pursuit/1
  kappa_des/1 -> Terminator2/1
  p_des/1 -> Switches/1(p_des)
  psi_des/1 -> Switches/2(psi_des)
  Pure Pursuit/1 -> Switches/6(lin_vel)
  Pure Pursuit/2 -> Switches/7(curvature)
  v_lim_des/1 -> Pure Pursuit/3
  Switches/1(ang_true) -> Outer Wheel Limiter/1(ang)
  Switches/2(vel_true) -> Outer Wheel Limiter/2(vel)
  Outer Wheel Limiter/1(m1_rate_cmd) -> m1_rate_cmd/1
  Outer Wheel Limiter/2(m2_rate_cmd) -> m2_rate_cmd/1

== system SHRKIM002_Dubins/Robot Navigation & Control/Trajectory Generator/Metrics ==
  index : Inport
  kappa_max : Inport  Port=2
  dk_max : Inport  Port=3
  n_jumps : Inport  Port=4
  Display : Display
  Display1 : Display
  Display2 : Display
  Terminator : Terminator
  wires:
  kappa_max/1 -> Display/1
  index/1 -> Terminator/1
  dk_max/1 -> Display1/1
  n_jumps/1 -> Display2/1

== system SHRKIM002_Dubins/Robot Navigation & Control/Feedback Controller/LMPC/LMPC Model ==
  Bus Creator : BusCreator  Inputs=8
  MATLAB Function : MATLAB Function  TreatAsAtomicUnit=on
  lmpc_model_bus : Outport
  wires:
  MATLAB Function/4(D) -> Bus Creator/4  "D"
  MATLAB Function/3(C) -> Bus Creator/3  "C"
  MATLAB Function/2(B) -> Bus Creator/2  "B"
  MATLAB Function/6(U) -> Bus Creator/6  "U"
  MATLAB Function/5(X) -> Bus Creator/5  "X"
  [kappa_des] -> MATLAB Function/2(kappa)
  MATLAB Function/7(Y) -> Bus Creator/7  "Y"
  MATLAB Function/1(A) -> Bus Creator/1  "A"
  MATLAB Function/8(DX) -> Bus Creator/8  "DX"
  Bus Creator/1 -> lmpc_model_bus/1
  [v_lim_des] -> MATLAB Function/1(v)

== system SHRKIM002_Dubins/Robot Navigation & Control/Feedback Controller/LMPC/Metrics ==
  e_lat : Inport
  e_psi : Inport  Port=2
  Abs : Abs  SaturateOnIntegerOverflow=off
  Abs1 : Abs  SaturateOnIntegerOverflow=off
  Constant : Constant  Value=0
  Constant1 : Constant  Value=0
  Display{,1..3} (4 alike) : Display
  MinMax Running Resettable : simulink/Math Operations/MinMax Running Resettable  Function=max  vinit=0.0
  MinMax Running Resettable1 : simulink/Math Operations/MinMax Running Resettable  Function=max  vinit=0.0
  RMS : dspstat3/RMS  run=on  directionMode=Each column  dimension=1  InputProcessing=Columns as channels (frame based)  reset_popup=None
  RMS1 : dspstat3/RMS  run=on  directionMode=Each column  dimension=1  InputProcessing=Columns as channels (frame based)  reset_popup=None
  rad2deg : Gain  Gain=180/pi
  wires:
  e_lat/1 -> Abs/1, RMS/1
  e_psi/1 -> rad2deg/1
  RMS/1 -> Display/1  "e_lat_rms"
  Abs/1 -> MinMax Running Resettable/1
  Constant/1 -> MinMax Running Resettable/2
  MinMax Running Resettable/1 -> Display1/1  "e_lat_max"
  MinMax Running Resettable1/1 -> Display3/1  "e_psi_max"
  Constant1/1 -> MinMax Running Resettable1/2
  Abs1/1 -> MinMax Running Resettable1/1
  rad2deg/1 -> Abs1/1, RMS1/1
  RMS1/1 -> Display2/1  "e_psi_rms"

== system SHRKIM002_Dubins/Robot Navigation & Control/Feedback Controller/LMPC/Target wheel speeds ==
  kappa_des : Inport
  v_lim_des : Inport  Port=2
  Gain : Gain  Gain=1/r_w
  Mux : Mux  Inputs=2
  Product : Product
  Sum : Sum  Inputs=|+-
  Sum1 : Sum  Inputs=|++
  kappa_ff : Gain  Gain=d/(2*r_w)
  dphi_target : Outport
  wires:
  v_lim_des/1 -> Gain/1, Product/2
  kappa_ff/1 -> Sum/2, Sum1/2  "w_ff"
  Product/1 -> kappa_ff/1
  Mux/1 -> dphi_target/1
  Gain/1 -> Sum1/1, Sum/1  "base_d_phi"
  Sum/1 -> Mux/1  "m1_rate_target"
  Sum1/1 -> Mux/2  "m2_rate_target"
  kappa_des/1 -> Product/1

== system SHRKIM002_Dubins/Robot Navigation & Control/Feedback Controller/NMPC/Metrics ==
  e_lat : Inport
  e_psi : Inport  Port=2
  Abs : Abs  SaturateOnIntegerOverflow=off
  Abs1 : Abs  SaturateOnIntegerOverflow=off
  Constant : Constant  Value=0
  Constant1 : Constant  Value=0
  Display{,1..3} (4 alike) : Display
  MinMax Running Resettable : simulink/Math Operations/MinMax Running Resettable  Function=max  vinit=0.0
  MinMax Running Resettable1 : simulink/Math Operations/MinMax Running Resettable  Function=max  vinit=0.0
  RMS : dspstat3/RMS  run=on  directionMode=Each column  dimension=1  InputProcessing=Columns as channels (frame based)  reset_popup=None
  RMS1 : dspstat3/RMS  run=on  directionMode=Each column  dimension=1  InputProcessing=Columns as channels (frame based)  reset_popup=None
  rad2deg : Gain  Gain=180/pi
  wires:
  e_lat/1 -> Abs/1, RMS/1
  e_psi/1 -> rad2deg/1
  RMS/1 -> Display/1  "e_lat_rms"
  Abs/1 -> MinMax Running Resettable/1
  Constant/1 -> MinMax Running Resettable/2
  MinMax Running Resettable/1 -> Display1/1  "e_lat_max"
  MinMax Running Resettable1/1 -> Display3/1  "e_psi_max"
  Constant1/1 -> MinMax Running Resettable1/2
  Abs1/1 -> MinMax Running Resettable1/1
  rad2deg/1 -> Abs1/1, RMS1/1
  RMS1/1 -> Display2/1  "e_psi_rms"

== system SHRKIM002_Dubins/Robot Navigation & Control/Feedback Controller/NMPC/Target wheel speeds ==
  kappa_des : Inport
  v_lim_des : Inport  Port=2
  Gain : Gain  Gain=1/r_w
  Mux : Mux  Inputs=2
  Product : Product
  Reshape : Reshape  OutputDimensionality=Row vector (2-D)
  Sum : Sum  Inputs=|+-
  Sum1 : Sum  Inputs=|++
  kappa_ff : Gain  Gain=d/(2*r_w)
  dphi_target : Outport
  wires:
  v_lim_des/1 -> Gain/1, Product/2
  kappa_ff/1 -> Sum/2, Sum1/2  "w_ff"
  Product/1 -> kappa_ff/1
  Gain/1 -> Sum1/1, Sum/1  "base_d_phi"
  Sum/1 -> Mux/1  "m1_rate_target"
  Sum1/1 -> Mux/2  "m2_rate_target"
  kappa_des/1 -> Product/1
  Mux/1 -> Reshape/1
  Reshape/1 -> dphi_target/1

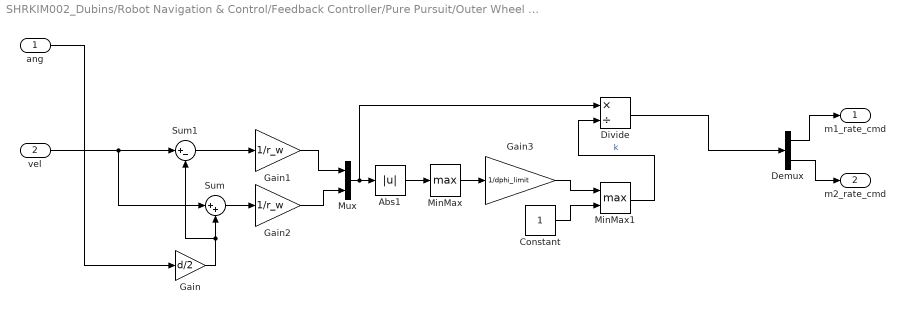
== system SHRKIM002_Dubins/Robot Navigation & Control/Feedback Controller/Pure Pursuit/Outer Wheel Limiter ==
  ang : Inport
  vel : Inport  Port=2
  Abs1 : Abs  SaturateOnIntegerOverflow=off
  Constant : Constant
  Demux : Demux  Outputs=2
  Divide : Product  Inputs=*/
  Gain : Gain  Gain=d/2
  Gain1 : Gain  Gain=1/r_w
  Gain2 : Gain  Gain=1/r_w
  Gain3 : Gain  Gain=1/dphi_limit
  MinMax : MinMax  Function=max
  MinMax1 : MinMax  Function=max  Inputs=2
  Mux : Mux  Inputs=2
  Sum : Sum  Inputs=|++
  Sum1 : Sum  Inputs=|+-
  m1_rate_cmd : Outport
  m2_rate_cmd : Outport  Port=2
  wires:
  Gain/1 -> Sum1/2, Sum/2
  Sum/1 -> Gain2/1
  Sum1/1 -> Gain1/1
  vel/1 -> Sum/1, Sum1/1
  ang/1 -> Gain/1
  Gain1/1 -> Mux/1
  MinMax/1 -> Gain3/1
  Gain2/1 -> Mux/2
  Mux/1 -> Divide/1, Abs1/1
  Abs1/1 -> MinMax/1
  Gain3/1 -> MinMax1/1
  Constant/1 -> MinMax1/2
  MinMax1/1 -> Divide/2  "k"
  Demux/1 -> m1_rate_cmd/1
  Demux/2 -> m2_rate_cmd/1
  Divide/1 -> Demux/1

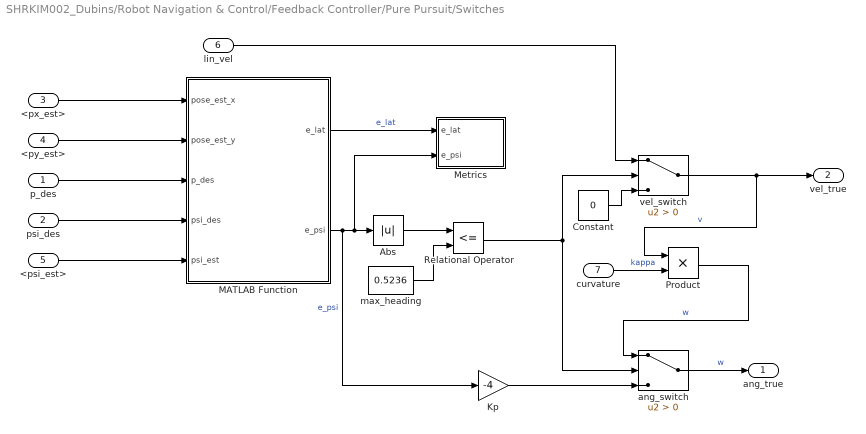
== system SHRKIM002_Dubins/Robot Navigation & Control/Feedback Controller/Pure Pursuit/Switches ==
  p_des : Inport
  psi_des : Inport  Port=2
  <px_est> : Inport  Port=3
  <py_est> : Inport  Port=4
  <psi_est> : Inport  Port=5
  lin_vel : Inport  Port=6
  curvature : Inport  Port=7
  Abs : Abs  SaturateOnIntegerOverflow=off
  Constant : Constant  Value=0
  Kp : Gain  Gain=-4
  MATLAB Function : MATLAB Function  TreatAsAtomicUnit=on
  Metrics : Subsystem
  Product : Product
  Relational Operator : RelationalOperator  Operator=<=  OutDataTypeStr=boolean  RndMeth=Simplest  InputSameDT=off
  ang_switch : Switch  Criteria=u2 > Threshold  SaturateOnIntegerOverflow=off  InputSameDT=off
  max_heading : Constant  Value=0.5236
  vel_switch : Switch  Criteria=u2 > Threshold  SaturateOnIntegerOverflow=off  InputSameDT=off
  ang_true : Outport
  vel_true : Outport  Port=2
  wires:
  Relational Operator/1 -> vel_switch/2, ang_switch/2
  vel_switch/1 -> Product/1, vel_true/1  "v"
  lin_vel/1 -> vel_switch/1
  Product/1 -> ang_switch/1  "w"
  Constant/1 -> vel_switch/3
  curvature/1 -> Product/2  "kappa"
  ang_switch/1 -> ang_true/1  "w"
  max_heading/1 -> Relational Operator/2
  Abs/1 -> Relational Operator/1
  <psi_est>/1 -> MATLAB Function/5(psi_est)
  MATLAB Function/1(e_lat) -> Metrics/1(e_lat)  "e_lat"
  <px_est>/1 -> MATLAB Function/1(pose_est_x)
  psi_des/1 -> MATLAB Function/4(psi_des)
  p_des/1 -> MATLAB Function/3(p_des)
  <py_est>/1 -> MATLAB Function/2(pose_est_y)
  MATLAB Function/2(e_psi) -> Kp/1, Metrics/2(e_psi), Abs/1  "e_psi"
  Kp/1 -> ang_switch/3

== system SHRKIM002_Dubins/Robot Navigation & Control/Feedback Controller/Pure Pursuit/Switches/Metrics ==
  e_lat : Inport
  e_psi : Inport  Port=2
  Abs : Abs  SaturateOnIntegerOverflow=off
  Abs1 : Abs  SaturateOnIntegerOverflow=off
  Constant : Constant  Value=0
  Constant1 : Constant  Value=0
  Display{,1..3} (4 alike) : Display
  MinMax Running Resettable : simulink/Math Operations/MinMax Running Resettable  Function=max  vinit=0.0
  MinMax Running Resettable1 : simulink/Math Operations/MinMax Running Resettable  Function=max  vinit=0.0
  RMS : dspstat3/RMS  run=on  directionMode=Each column  dimension=1  InputProcessing=Columns as channels (frame based)  reset_popup=None
  RMS1 : dspstat3/RMS  run=on  directionMode=Each column  dimension=1  InputProcessing=Columns as channels (frame based)  reset_popup=None
  rad2deg : Gain  Gain=180/pi
  wires:
  e_lat/1 -> Abs/1, RMS/1
  e_psi/1 -> rad2deg/1
  RMS/1 -> Display/1  "e_lat_rms"
  Abs/1 -> MinMax Running Resettable/1
  Constant/1 -> MinMax Running Resettable/2
  MinMax Running Resettable/1 -> Display1/1  "e_lat_max"
  MinMax Running Resettable1/1 -> Display3/1  "e_psi_max"
  Constant1/1 -> MinMax Running Resettable1/2
  Abs1/1 -> MinMax Running Resettable1/1
  rad2deg/1 -> Abs1/1, RMS1/1
  RMS1/1 -> Display2/1  "e_psi_rms"

== matlab function SHRKIM002_Dubins/Robot Navigation & Control/Feedback Controller/LMPC/Lateral Error Calculation ==
  data: pose_est_x input; pose_est_y input; e_lat output; p_des input; psi_des input; psi_est input; e_psi output
function [e_lat, e_psi] = calc_error(pose_est_x, pose_est_y, p_des, psi_des, psi_est)

    % Global difference
    dx = pose_est_x - p_des(1);
    dy = pose_est_y - p_des(2);
    
    % Local (path bound) lateral difference
    e_lat = -sin(psi_des) * dx + cos(psi_des) * dy;

    e_psi = atan2(sin(psi_est-psi_des),cos(psi_est - psi_des));
end

== matlab function SHRKIM002_Dubins/2Wh. Robot/MATLAB Function1 ==
  data: pose_est input; p_des_array input; ts input; track_width parameter
function robotVisualiser(pose_est, p_des_array, ts, track_width)

    coder.extrinsic('fill', 'set', 'figure', 'shg', 'axis', 'hold', 'grid','legend', 'drawnow', 'getframe', 'frame2im', 'rgb2ind', 'imwrite', 'subplot', 'clf', 'sgtitle', 'axes');
    % Persistent variable keeps the plot handle so it doesn't flicker
    persistent h1 h2 h3 h4 hh1 hh2 hh3 hh4 index;

    if( isempty(index) )
        index = 1;
    end

    %Est pose
    x = pose_est(1);
    y = pose_est(2);
    th = pose_est(3);

    % Est pose triangle
    r = 0.2; 
    px_ = [x + r*cos(th), x + r*cos(th+2.5), x + r*cos(th-2.5), x + r*cos(th)];
    py_ = [y + r*sin(th), y + r*sin(th+2.5), y + r*sin(th-2.5), y + r*sin(th)];

    lim_overview = [min(p_des_array(1,:)) - track_width, max(p_des_array(1,:)) + track_width, min(p_des_array(2,:)) - track_width, max(p_des_array(2,:)) + track_width];

    zoom_size = 2.0; % Adjust this value to zoom in/out closer to the robot (in meters)
    lim_closeup  = [x - zoom_size, x + zoom_size, y - zoom_size, y + zoom_size];

    % If first time, create the plot. Otherwise, update data.
    if isempty(h1) || isempty(hh2) || isempty(h3) || isempty(h4) || isempty(hh1)

        half_w = track_width/2;
        n = size(p_des_array,2);
        l_bound = zeros(2, n);
        r_bound = zeros(2, n);

        % checking if the first and last waypoint are effectively in the same spot
        closed = norm(p_des_array(:,1) - p_des_array(:,n)) < 1e-9;

        for i = 1:n
            i_prev = i-1;
            i_next = i+1;

            if i == 1
                if closed
                    i_prev = n-1;
                else 
                    i_prev = 1;
                end
            end 

            if i == n
                if closed
                    i_next = 2;
                else
                    i_next = n;
                end
            end

            % tangent vector at each point
            vect = p_des_array(:,i_next) - p_des_array(:,i_prev);
            n_vect = norm(vect);

            % Making the tangent vector a unit vector
            % Point robot at track
            if n_vect < 1e-12
                dir_vec = p_des_array(:, 2) - p_des_array(:, 1);
                u_vect = dir_vec / norm(dir_vec);
            else
                u_vect = vect/n_vect;
            end

            % normal vector at each point
            norm_vect = [-u_vect(2); u_vect(1)];
            l_bound(:, i) = p_des_array(:,i) + half_w*norm_vect;
            r_bound(:, i) = p_des_array(:,i) - half_w*norm_vect;

        end 

        fig = figure(1);           % Assigns a specific ID to the window
        set(fig, 'Visible', 'on', 'Position', [100, 100, 1000, 550]); % wider window to fit everything
        shg;                       % "Show Graph" - brings the window to the front
        clf(fig);

        % left subplot of full track overview
        subplot('Position', [0.06, 0.12, 0.36, 0.78]);
        hold off;
        h1 = fill(px_, py_, 'g', 'LineWidth', 1);
        hold on;
        %h2 = plot(p_des_array(1,:),p_des_array(2,:),'--k',MarkerFaceColor='k');
        h3 = plot(l_bound(1,:),  l_bound(2,:),  '-k', 'LineWidth',1);
        h4 = plot(r_bound(1,:), r_bound(2,:), '-k', 'LineWidth',1);
        %legend('Robot','Centerline', 'Track Limit', Location='northeast');
        grid on;
        axis equal;
        axis(lim_overview);
        title('Track Overview');

        % right subplot of zoomed view
        subplot('Position', [0.58, 0.12, 0.36, 0.78]);
        hold off;
        hh1 = fill(px_, py_, 'g', 'LineWidth', 1);
        hold on;
        hh2 = plot(p_des_array(1,:), p_des_array(2,:), '--k', 'MarkerFaceColor', 'k');
        hh3 = plot(l_bound(1,:), l_bound(2,:), '-k', 'LineWidth', 1);
        hh4 = plot(r_bound(1,:), r_bound(2,:), '-k', 'LineWidth', 1);
        grid on;
        axis equal;
        axis(lim_closeup);
        title('Robot Tracking View');

        % shared legend
        h_leg = legend([h1, hh2, h3], {'Robot', 'Centerline', 'Track Limit'});
        set(h_leg, 'Position', [0.40, 0.4, 0.14, 0.2], 'Units', 'normalized');

    else

        % update overview
        subplot('Position', [0.06, 0.12, 0.36, 0.78]);
        set(h1, 'XData', px_, 'YData', py_);
        %set(h2, 'XData', p_des_array(1,:), 'YData', p_des_array(2,:));
        axis(lim_overview);
        title('Track Overview');

        % update close up
        subplot('Position', [0.58, 0.12, 0.36, 0.78]);
        set(hh1, 'XData', px_, 'YData', py_);
        set(hh2, 'XData', p_des_array(1,:), 'YData', p_des_array(2,:));
        axis(lim_closeup);

    end

    % shared title
    sgtitle(['Robot Lap Time: ', num2str(ts), ' s'], 'FontSize', 12, 'FontWeight', 'bold');

    drawnow limitrate; % High-speed update

    % create gif to be saved
    gif_filename = 'robot_track_simulation.gif';
    sample_rate = 15; % Capture 1 frame every 15 steps 
    delay_time  = 0.1; % Frame duration in seconds (0.1s = 10 FPS playback)

    if mod(index, sample_rate) == 0
        % Capture frame from current figure
        frame = getframe(figure(1));
        im = frame2im(frame);
        [imind, cm] = rgb2ind(im, 256);

        % Write first frame or append subsequent frames
        if index == sample_rate
            imwrite(imind, cm, gif_filename, 'gif', 'Loopcount', inf, 'DelayTime', delay_time);
        else
            imwrite(imind, cm, gif_filename, 'gif', 'WriteMode', 'append', 'DelayTime', delay_time);
        end
    end

    index = index + 1;
end

== matlab function SHRKIM002_Dubins/Robot Navigation & Control/MATLAB Function ==
  data: waypoints output; wp input
function waypoints = centerlineTrack(wp)
    waypoints = wp;
end

== matlab function SHRKIM002_Dubins/Robot Navigation & Control/Feedback Controller/LMPC/LMPC Model/MATLAB Function ==
  data: v input; A output; kappa input; B output; C output; D output; X output; U output; Y output; DX output; r_w parameter; d parameter; sample_f parameter
function [A,B,C,D,X,U,Y,DX] = lmpc_model(v, kappa, r_w, d, sample_f)

Ts = 1/sample_f;

% effect of left (1) and right (2) wheel on de_psi
b1 = -r_w/d - kappa*r_w/2;
b2 =  r_w/d - kappa*r_w/2;

% states [e_lat; e_psi]

A  = [1 v*Ts; 0 1]; 
B  = [v*Ts^2/2*b1, v*Ts^2/2*b2;
      Ts*b1,       Ts*b2];
C  = eye(2);  D = zeros(2);

X  = zeros(2,1); 
U = zeros(2,1); 
Y = zeros(2,1); 
DX = zeros(2,1);
end

== matlab function SHRKIM002_Dubins/Robot Navigation & Control/Pose Estimator/MATLAB Function ==
  settings: updateMethod=DISCRETE  sampleTime=0.02
  data: v input; px_est output; psi_dot input; py_est output; psi_est output; dT input; pose_est_xy output; waypoints input
function [px_est, py_est, psi_est, pose_est_xy] = poseEstimator(v, psi_dot, dT, waypoints)

persistent T
if( isempty(T) )
    % at start find waypoints to set starting angle

    % use first and fifth waypoint
    w1 = waypoints(:,1);
    w2 = waypoints(:,5);

    % initial heading angle
    psi_init = atan2(w2(2) - w1(2), w2(1) - w1(1));

    % transformation matrix to start set to face the track
    T = [cos(psi_init), -sin(psi_init), w1(1);
        sin(psi_init), cos(psi_init), w1(2);
        0, 0, 1];
end


delta_psi = psi_dot * dT;

% checking if the angle is big enough so that there is no dividing by 0 error
if abs(psi_dot) > 1e-4

    R = [cos(delta_psi), -sin(delta_psi);
        sin(delta_psi),  cos(delta_psi)];

    J = [sin(delta_psi)/delta_psi,     (cos(delta_psi)-1)/delta_psi;
        (1-cos(delta_psi))/delta_psi, sin(delta_psi)/delta_psi];

    T_inc = [R, J*[v; 0]*dT; 0, 0 ,1];
    
else 
    T_inc = [cos(delta_psi), -sin(delta_psi), v * cos(delta_psi) * dT; 
             sin(delta_psi),  cos(delta_psi), v * sin(delta_psi) * dT;
             0 0 1];
end 

T = T*T_inc;

px_est  = T(1, 3);
py_est  = T(2, 3);
psi_est = atan2(T(2,1),T(1,1));
pose_est_xy = [px_est; py_est];

end

== matlab function SHRKIM002_Dubins/2Wh. Robot/2Wh. Kinematics/MATLAB Function ==
  settings: updateMethod=DISCRETE
  data: waypoints input; dpx input; dpsi input; t output; psi output
function [t,psi] = updatePose(waypoints, dpx, dpsi)

persistent T;

if( isempty(T) )
    % at start find waypoints to set starting angle

    % use first and fifth waypoint
    w1 = waypoints(:,1);
    w2 = waypoints(:,5);

    % initial heading angle
    psi_init = atan2(w2(2) - w1(2), w2(1) - w1(1));

    % transformation matrix to start set to face the track
    T = [cos(psi_init), -sin(psi_init), w1(1);
        sin(psi_init), cos(psi_init), w1(2);
        0, 0, 1];
end

R = [cos(dpsi) -sin(dpsi);
      sin(dpsi)  cos(dpsi)];

if( abs(dpsi)<1e-5 )
    J = eye(2);
else
    J = [sin(dpsi)/(dpsi)     (cos(dpsi)-1)/(dpsi);
        (1-cos(dpsi))/(dpsi) sin(dpsi)/(dpsi)   ];
end

T_inc = [R J*[dpx 0]'; 0 0 1]; 
T = T*T_inc;

t = T(1:2,3);
psi = atan2(T(2,1),T(1,1));
end

== matlab function SHRKIM002_Dubins/Robot Navigation & Control/Feedback Controller/Pure Pursuit/Switches/MATLAB Function ==
  data: pose_est_x input; e_lat output; pose_est_y input; p_des input; psi_des input; psi_est input; e_psi output
function [e_lat, e_psi] = calc_error(pose_est_x, pose_est_y, p_des, psi_des, psi_est)
    
% Global difference
    dx = pose_est_x - p_des(1);
    dy = pose_est_y - p_des(2);
    
    % Local (path bound) lateral difference
    e_lat = -sin(psi_des) * dx + cos(psi_des) * dy;
    
    % Properly wrapped heading error
    e_psi = atan2(sin(psi_est - psi_des), cos(psi_est - psi_des));
end

== matlab function SHRKIM002_Dubins/Robot Navigation & Control/Feedback Controller/NMPC/Lateral Error Calculation ==
  data: pose_est_x input; pose_est_y input; e_lat output; p_des input; psi_des input; psi_est input; e_psi output
function [e_lat, e_psi] = calc_error(pose_est_x, pose_est_y, p_des, psi_des, psi_est)

    % Global difference
    dx = pose_est_x - p_des(1);
    dy = pose_est_y - p_des(2);
    
    % Local (path bound) lateral difference
    e_lat = -sin(psi_des) * dx + cos(psi_des) * dy;

    e_psi = atan2(sin(psi_est-psi_des),cos(psi_est - psi_des));
end
